simulink model "XFLUID04_reference"  (R2025a)
settings: Solver=ode23t  StartTime=0  StopTime=20  MaxStep=0.02  RelTol=1e-3  AbsTol=1e-4  EnableMultiTasking=on
PreLoadFcn:
  | warning('off','Simulink:Commands:LoadMdlParameterizedLink');
PostLoadFcn:
  | warning off sm:compiler:topologyAnalysis:DanglingBlock
  | warning off Simulink:SL_SolverMaskedZC;
  | warning off Simulink:SL_SolverIgnoredZCBracketing;
  | warning off Simulink:Engine:SolverMinStepNonlinearIterWarnForDAE;
  | warning off simscape:compiler:sli:init:SolverNotRecommended
  | warning off Simulink:Engine:UsingDiscreteSolver
  | warning('off','sm:sli:setup:compile:LocalSolverNotSupported')
  | warning off physmod:simscape:compiler:sli:init:SolverNotRecommended
  | warning off sm:sli:visualization:ModelRefNotSupported
  | warning off Simulink:modelReference:ProtectedModelCallbackLostWarning
StartFcn:
  | tic;
StopFcn:
  | Elapsed_Sim_Time = toc;
  | disp(['Elapsed Sim Time = ' num2str(Elapsed_Sim_Time)]);
undefined symbols (not defined in the file): actuator_hs_b, actuator_hs_k, lift_target_mm, Local, motion_start_s, motor_damping, pressure_step_offset_s, ramp_duration_s, Scissor_Lift_Param, supply_pressure_bar, supply_pressure_step_fraction, target_hold_s, X, Y, Z
libraries: fl_lib x108, sm_lib x41, Scissor_Parts_Lib x24, nesl_utility x9, SimscapeFluids_lib x2, Custom_lib x2, slpidlib x1, fl_ps_legacy_lib x1, simulink x1, ee_lib x1, Motor_Lib x1, sdl_lib x1
(part 3 of 3)

== system XFLUID04_reference/Load/Scissor/Base/Platform ==
  Block R : Scissor_Parts_Lib/Block  L=Scissor_Lift_Param.Upper_Platform.Length  W=Scissor_Lift_Param.Upper_Platform.Width  H=Scissor_Lift_Param.Upper_Platform.Height  z_ori=Local +Z  rho=Scissor_Lift_Param.Upper_Platform.Density  clr=Scissor_Lift_Param.Upper_Platform.Color  opc=Scissor_Lift_Param.Upper_Platform.Opacity
  Transform Orientation : sm_lib/Frames and Transforms/Rigid Transform  RotationMethod=StandardAxis  FollAlignAxisA=+X  BaseAlignAxisA=+Y  FollAlignAxisB=+Y  BaseAlignAxisB=+Z  RotationStandardAxis=+X  RotationAngle=90  RotationAngleUnits=deg  RotationArbitraryAxis=[0 0 1]  RotationSequenceAxes=FollowerAxes  RotationSequence=XYX  RotationSequenceAngles=[0 0 0]  RotationSequenceAnglesUnits=deg  RotationMatrix=[1 0 0; 0 1 0; 0 0 1]  Quaternion=[1 0 0 0]  TranslationMethod=None  TranslationCartesianOffset=[0 0 0]  TranslationCartesianOffsetUnits=m  TranslationStandardAxis=+X  TranslationStandardOffset=0  TranslationStandardOffsetUnits=m  TranslationROffset=0  TranslationROffsetUnits=m  TranslationThetaOffset=0  TranslationThetaOffsetUnits=deg  TranslationZOffset=0  TranslationZOffsetUnits=m
  Transform Platform CG : sm_lib/Frames and Transforms/Rigid Transform  RotationMethod=StandardAxis  FollAlignAxisA=+X  BaseAlignAxisA=+Y  FollAlignAxisB=+Y  BaseAlignAxisB=+Z  RotationStandardAxis=+Y  RotationAngle=90  RotationAngleUnits=deg  RotationArbitraryAxis=[0 0 1]  RotationSequenceAxes=FollowerAxes  RotationSequence=XYX  RotationSequenceAngles=[0 0 0]  RotationSequenceAnglesUnits=deg  RotationMatrix=[1 0 0; 0 1 0; 0 0 1]  Quaternion=[1 0 0 0]  TranslationMethod=StandardAxis  TranslationCartesianOffset=[0 0 0]  TranslationCartesianOffsetUnits=cm  TranslationStandardAxis=-X  TranslationStandardOffset=Scissor_Lift_Param.Link.Length  TranslationStandardOffsetUnits=cm  TranslationROffset=0  TranslationROffsetUnits=m  TranslationThetaOffset=0  TranslationThetaOffsetUnits=deg  TranslationZOffset=0  TranslationZOffsetUnits=m
  Transform Platform CP : sm_lib/Frames and Transforms/Rigid Transform  RotationMethod=None  FollAlignAxisA=+X  BaseAlignAxisA=+Y  FollAlignAxisB=+Y  BaseAlignAxisB=+Z  RotationStandardAxis=+Y  RotationAngle=0  RotationAngleUnits=deg  RotationArbitraryAxis=[0 0 1]  RotationSequenceAxes=FollowerAxes  RotationSequence=XYX  RotationSequenceAngles=[0 0 0]  RotationSequenceAnglesUnits=deg  RotationMatrix=[1 0 0; 0 1 0; 0 0 1]  Quaternion=[1 0 0 0]  TranslationMethod=Cartesian  TranslationCartesianOffset=[0 -Scissor_Lift_Param.Upper_Platform.Height/2 0]  TranslationCartesianOffsetUnits=cm  TranslationStandardAxis=-Y  TranslationStandardOffset=Scissor_Lift_Param.Roller.Roller_Radius  TranslationStandardOffsetUnits=cm  TranslationROffset=0  TranslationROffsetUnits=m  TranslationThetaOffset=0  TranslationThetaOffsetUnits=deg  TranslationZOffset=0  TranslationZOffsetUnits=m
  S : PMIOPort  Side=Right
  W : PMIOPort  Port=2  Side=Left
  connections:
  Block R/LConn1 -- Transform Platform CG/RConn1
  Transform Platform CP/RConn1 -- Transform Orientation/RConn1 -- Transform Platform CG/LConn1
  Transform Orientation/LConn1 -- W/RConn1
  Transform Platform CP/LConn1 -- S/RConn1

== system XFLUID04_reference/Load/Scissor/Base/Rear Shaft ==
  Blocks L : Scissor_Parts_Lib/Base Blocks  block_length=Scissor_Lift_Param.Base_Block.Length  block_width=Scissor_Lift_Param.Base_Block.Width  block_height=Scissor_Lift_Param.Base_Block.Height  shaft_radius=Scissor_Lift_Param.Roller.Shaft_Radius  shaft_length=Scissor_Lift_Param.Roller.Shaft_Length  material_density=Scissor_Lift_Param.Base_Block.Density  material_color=Scissor_Lift_Param.Base_Block.Color  material_opacity=Scissor_Lift_Param.Base_Block.Opacity
  Blocks R : Scissor_Parts_Lib/Base Blocks  block_length=Scissor_Lift_Param.Base_Block.Length  block_width=Scissor_Lift_Param.Base_Block.Width  block_height=Scissor_Lift_Param.Base_Block.Height  shaft_radius=Scissor_Lift_Param.Roller.Shaft_Radius  shaft_length=Scissor_Lift_Param.Roller.Shaft_Length  material_density=Scissor_Lift_Param.Base_Block.Density  material_color=Scissor_Lift_Param.Base_Block.Color  material_opacity=Scissor_Lift_Param.Base_Block.Opacity
  Shaft L : Scissor_Parts_Lib/Shaft  L=Scissor_Lift_Param.Base_Act_Shaft.Length/2  r=Scissor_Lift_Param.Base_Act_Shaft.Radius  theta=0  z_ori=Local +Z  Ro=Scissor_Lift_Param.Base_Act_Shaft.Density  clr=Scissor_Lift_Param.Base_Act_Shaft.Color  opc=Scissor_Lift_Param.Base_Act_Shaft.Opacity
  Shaft R : Scissor_Parts_Lib/Shaft  L=Scissor_Lift_Param.Base_Act_Shaft.Length/2  r=Scissor_Lift_Param.Base_Act_Shaft.Radius  theta=0  z_ori=Local +Z  Ro=Scissor_Lift_Param.Base_Act_Shaft.Density  clr=Scissor_Lift_Param.Base_Act_Shaft.Color  opc=Scissor_Lift_Param.Base_Act_Shaft.Opacity
  Transform Base Shaft : sm_lib/Frames and Transforms/Rigid Transform  RotationMethod=None  FollAlignAxisA=+X  BaseAlignAxisA=+Y  FollAlignAxisB=+Y  BaseAlignAxisB=+Z  RotationStandardAxis=+Y  RotationAngle=0  RotationAngleUnits=deg  RotationArbitraryAxis=[0 0 1]  RotationSequenceAxes=FollowerAxes  RotationSequence=XYX  RotationSequenceAngles=[0 0 0]  RotationSequenceAnglesUnits=deg  RotationMatrix=[1 0 0; 0 1 0; 0 0 1]  Quaternion=[1 0 0 0]  TranslationMethod=Cartesian  TranslationCartesianOffset=[0 -Scissor_Lift_Param.Base_Block.Height/2 0]  TranslationCartesianOffsetUnits=cm  TranslationStandardAxis=-Y  TranslationStandardOffset=Scissor_Lift_Param.Roller.Roller_Radius  TranslationStandardOffsetUnits=cm  TranslationROffset=0  TranslationROffsetUnits=m  TranslationThetaOffset=0  TranslationThetaOffsetUnits=deg  TranslationZOffset=0  TranslationZOffsetUnits=m
  Transform C to L : sm_lib/Frames and Transforms/Rigid Transform  RotationMethod=None  FollAlignAxisA=+X  BaseAlignAxisA=+Y  FollAlignAxisB=+Y  BaseAlignAxisB=+Z  RotationStandardAxis=+X  RotationAngle=90  RotationAngleUnits=deg  RotationArbitraryAxis=[0 0 1]  RotationSequenceAxes=FollowerAxes  RotationSequence=XYX  RotationSequenceAngles=[0 0 0]  RotationSequenceAnglesUnits=deg  RotationMatrix=[1 0 0; 0 1 0; 0 0 1]  Quaternion=[1 0 0 0]  TranslationMethod=StandardAxis  TranslationCartesianOffset=[0 0 0]  TranslationCartesianOffsetUnits=cm  TranslationStandardAxis=+Z  TranslationStandardOffset=Scissor_Lift_Param.Link_Separation.Outer_Outer/2  TranslationStandardOffsetUnits=cm  TranslationROffset=0  TranslationROffsetUnits=m  TranslationThetaOffset=0  TranslationThetaOffsetUnits=deg  TranslationZOffset=0  TranslationZOffsetUnits=m
  Transform C to R : sm_lib/Frames and Transforms/Rigid Transform  RotationMethod=None  FollAlignAxisA=+X  BaseAlignAxisA=+Y  FollAlignAxisB=+Y  BaseAlignAxisB=+Z  RotationStandardAxis=+X  RotationAngle=90  RotationAngleUnits=deg  RotationArbitraryAxis=[0 0 1]  RotationSequenceAxes=FollowerAxes  RotationSequence=XYX  RotationSequenceAngles=[0 0 0]  RotationSequenceAnglesUnits=deg  RotationMatrix=[1 0 0; 0 1 0; 0 0 1]  Quaternion=[1 0 0 0]  TranslationMethod=StandardAxis  TranslationCartesianOffset=[0 0 0]  TranslationCartesianOffsetUnits=cm  TranslationStandardAxis=-Z  TranslationStandardOffset=Scissor_Lift_Param.Link_Separation.Outer_Outer/2  TranslationStandardOffsetUnits=cm  TranslationROffset=0  TranslationROffsetUnits=m  TranslationThetaOffset=0  TranslationThetaOffsetUnits=deg  TranslationZOffset=0  TranslationZOffsetUnits=m
  R : PMIOPort  Side=Right
  P : PMIOPort  Port=2  Side=Left
  connections:
  Transform C to R/LConn1 -- Transform Base Shaft/RConn1 -- Transform C to L/LConn1 -- P/RConn1
  Blocks L/LConn1 -- Transform C to L/RConn1
  Shaft R/RConn1 -- Transform Base Shaft/LConn1 -- Shaft L/LConn1 -- R/RConn1
  Blocks R/LConn1 -- Transform C to R/RConn1

== system XFLUID04_reference/Load/Scissor/Inner Links/Link Connect ==
  Transform Outer FC : sm_lib/Frames and Transforms/Rigid Transform  RotationMethod=None  FollAlignAxisA=+X  BaseAlignAxisA=+Y  FollAlignAxisB=+Y  BaseAlignAxisB=+Z  RotationStandardAxis=+Z  RotationAngle=0  RotationAngleUnits=deg  RotationArbitraryAxis=[0 0 1]  RotationSequenceAxes=FollowerAxes  RotationSequence=XYX  RotationSequenceAngles=[0 0 0]  RotationSequenceAnglesUnits=deg  RotationMatrix=[1 0 0; 0 1 0; 0 0 1]  Quaternion=[1 0 0 0]  TranslationMethod=StandardAxis  TranslationCartesianOffset=[0 0 0]  TranslationCartesianOffsetUnits=cm  TranslationStandardAxis=+Z  TranslationStandardOffset=Scissor_Lift_Param.Link_Separation.Inner_Inner/2  TranslationStandardOffsetUnits=cm  TranslationROffset=0  TranslationROffsetUnits=m  TranslationThetaOffset=0  TranslationThetaOffsetUnits=deg  TranslationZOffset=0  TranslationZOffsetUnits=m
  Transform Outer FL : sm_lib/Frames and Transforms/Rigid Transform  RotationMethod=None  FollAlignAxisA=+X  BaseAlignAxisA=+Y  FollAlignAxisB=+Y  BaseAlignAxisB=+Z  RotationStandardAxis=+Z  RotationAngle=0  RotationAngleUnits=deg  RotationArbitraryAxis=[0 0 1]  RotationSequenceAxes=FollowerAxes  RotationSequence=XYX  RotationSequenceAngles=[0 0 0]  RotationSequenceAnglesUnits=deg  RotationMatrix=[1 0 0; 0 1 0; 0 0 1]  Quaternion=[1 0 0 0]  TranslationMethod=StandardAxis  TranslationCartesianOffset=[0 0 0]  TranslationCartesianOffsetUnits=cm  TranslationStandardAxis=+Z  TranslationStandardOffset=Scissor_Lift_Param.Link_Separation.Inner_Inner/2  TranslationStandardOffsetUnits=cm  TranslationROffset=0  TranslationROffsetUnits=m  TranslationThetaOffset=0  TranslationThetaOffsetUnits=deg  TranslationZOffset=0  TranslationZOffsetUnits=m
  L : PMIOPort  Side=Right
  C : PMIOPort  Port=2  Side=Left
  R : PMIOPort  Port=3  Side=Right
  connections:
  Transform Outer FL/LConn1 -- C/RConn1 -- Transform Outer FC/RConn1
  Transform Outer FC/LConn1 -- R/RConn1
  Transform Outer FL/RConn1 -- L/RConn1

== system XFLUID04_reference/Load/Scissor/Inner Links/Rollers ==
  Roller L : Scissor_Parts_Lib/Base Roller  roller_length=Scissor_Lift_Param.Roller.Roller_Length  roller_radius=Scissor_Lift_Param.Roller.Roller_Radius  shaft_length=Scissor_Lift_Param.Roller.Shaft_Length  shaft_radius=Scissor_Lift_Param.Roller.Shaft_Radius  material_density=Scissor_Lift_Param.Roller.Density  material_color=Scissor_Lift_Param.Roller.Color  material_opacity=Scissor_Lift_Param.Roller.Opacity
  Roller R : Scissor_Parts_Lib/Base Roller  roller_length=Scissor_Lift_Param.Roller.Roller_Length  roller_radius=Scissor_Lift_Param.Roller.Roller_Radius  shaft_length=Scissor_Lift_Param.Roller.Shaft_Length  shaft_radius=Scissor_Lift_Param.Roller.Shaft_Radius  material_density=Scissor_Lift_Param.Roller.Density  material_color=Scissor_Lift_Param.Roller.Color  material_opacity=Scissor_Lift_Param.Roller.Opacity
  Transform C to L : sm_lib/Frames and Transforms/Rigid Transform  RotationMethod=None  FollAlignAxisA=+X  BaseAlignAxisA=+Y  FollAlignAxisB=+Y  BaseAlignAxisB=+Z  RotationStandardAxis=+X  RotationAngle=90  RotationAngleUnits=deg  RotationArbitraryAxis=[0 0 1]  RotationSequenceAxes=FollowerAxes  RotationSequence=XYX  RotationSequenceAngles=[0 0 0]  RotationSequenceAnglesUnits=deg  RotationMatrix=[1 0 0; 0 1 0; 0 0 1]  Quaternion=[1 0 0 0]  TranslationMethod=StandardAxis  TranslationCartesianOffset=[0 0 0]  TranslationCartesianOffsetUnits=cm  TranslationStandardAxis=+Z  TranslationStandardOffset=Scissor_Lift_Param.Link_Separation.Inner_Inner/2  TranslationStandardOffsetUnits=cm  TranslationROffset=0  TranslationROffsetUnits=m  TranslationThetaOffset=0  TranslationThetaOffsetUnits=deg  TranslationZOffset=0  TranslationZOffsetUnits=m
  Transform C to R : sm_lib/Frames and Transforms/Rigid Transform  RotationMethod=None  FollAlignAxisA=+X  BaseAlignAxisA=+Y  FollAlignAxisB=+Y  BaseAlignAxisB=+Z  RotationStandardAxis=+X  RotationAngle=90  RotationAngleUnits=deg  RotationArbitraryAxis=[0 0 1]  RotationSequenceAxes=FollowerAxes  RotationSequence=XYX  RotationSequenceAngles=[0 0 0]  RotationSequenceAnglesUnits=deg  RotationMatrix=[1 0 0; 0 1 0; 0 0 1]  Quaternion=[1 0 0 0]  TranslationMethod=StandardAxis  TranslationCartesianOffset=[0 0 0]  TranslationCartesianOffsetUnits=cm  TranslationStandardAxis=-Z  TranslationStandardOffset=Scissor_Lift_Param.Link_Separation.Inner_Inner/2  TranslationStandardOffsetUnits=cm  TranslationROffset=0  TranslationROffsetUnits=m  TranslationThetaOffset=0  TranslationThetaOffsetUnits=deg  TranslationZOffset=0  TranslationZOffsetUnits=m
  Transform Lower P : sm_lib/Frames and Transforms/Rigid Transform  RotationMethod=StandardAxis  FollAlignAxisA=+X  BaseAlignAxisA=+Y  FollAlignAxisB=+Y  BaseAlignAxisB=+Z  RotationStandardAxis=+Y  RotationAngle=-90  RotationAngleUnits=deg  RotationArbitraryAxis=[0 0 1]  RotationSequenceAxes=FollowerAxes  RotationSequence=XYX  RotationSequenceAngles=[0 0 0]  RotationSequenceAnglesUnits=deg  RotationMatrix=[1 0 0; 0 1 0; 0 0 1]  Quaternion=[1 0 0 0]  TranslationMethod=Cartesian  TranslationCartesianOffset=[0 Scissor_Lift_Param.Base_Block.Height/2 0]  TranslationCartesianOffsetUnits=cm  TranslationStandardAxis=-Y  TranslationStandardOffset=Scissor_Lift_Param.Roller.Roller_Radius  TranslationStandardOffsetUnits=cm  TranslationROffset=0  TranslationROffsetUnits=m  TranslationThetaOffset=0  TranslationThetaOffsetUnits=deg  TranslationZOffset=0  TranslationZOffsetUnits=m
  S : PMIOPort  Side=Right
  LP : PMIOPort  Port=2  Side=Left
  connections:
  Roller L/RConn1 -- Transform C to L/RConn1
  Transform C to L/LConn1 -- Transform C to R/LConn1 -- Transform Lower P/RConn1 -- S/RConn1
  Roller R/RConn1 -- Transform C to R/RConn1
  Transform Lower P/LConn1 -- LP/RConn1

== system XFLUID04_reference/Load/Scissor/Inner Links/Shaft Actuator ==
  Shaft L : Scissor_Parts_Lib/Shaft  L=Scissor_Lift_Param.Link_Act_Shaft.Length/2  r=Scissor_Lift_Param.Link_Act_Shaft.Radius  theta=0  z_ori=Local +Z  Ro=Scissor_Lift_Param.Link_Act_Shaft.Density  clr=Scissor_Lift_Param.Colors.Yellow  opc=Scissor_Lift_Param.Link_Act_Shaft.Opacity
  Shaft R : Scissor_Parts_Lib/Shaft  L=Scissor_Lift_Param.Link_Act_Shaft.Length/2  r=Scissor_Lift_Param.Link_Act_Shaft.Radius  theta=0  z_ori=Local +Z  Ro=Scissor_Lift_Param.Link_Act_Shaft.Density  clr=Scissor_Lift_Param.Colors.Yellow  opc=Scissor_Lift_Param.Link_Act_Shaft.Opacity
  Transform Act Shaft : sm_lib/Frames and Transforms/Rigid Transform  RotationMethod=None  FollAlignAxisA=+X  BaseAlignAxisA=+Y  FollAlignAxisB=+Y  BaseAlignAxisB=+Z  RotationStandardAxis=+X  RotationAngle=90  RotationAngleUnits=deg  RotationArbitraryAxis=[0 0 1]  RotationSequenceAxes=FollowerAxes  RotationSequence=XYX  RotationSequenceAngles=[0 0 0]  RotationSequenceAnglesUnits=deg  RotationMatrix=[1 0 0; 0 1 0; 0 0 1]  Quaternion=[1 0 0 0]  TranslationMethod=StandardAxis  TranslationCartesianOffset=[0 0 0]  TranslationCartesianOffsetUnits=cm  TranslationStandardAxis=-X  TranslationStandardOffset=Scissor_Lift_Param.Link_Act_Shaft.Offset  TranslationStandardOffsetUnits=cm  TranslationROffset=0  TranslationROffsetUnits=m  TranslationThetaOffset=0  TranslationThetaOffsetUnits=deg  TranslationZOffset=0  TranslationZOffsetUnits=m
  Act : PMIOPort  Side=Right
  UP : PMIOPort  Port=2  Side=Left
  connections:
  Shaft R/RConn1 -- Shaft L/LConn1 -- Transform Act Shaft/RConn1 -- Act/RConn1
  Transform Act Shaft/LConn1 -- UP/RConn1

== system XFLUID04_reference/Load/Scissor/Outer Links/Rollers ==
  Roller L : Scissor_Parts_Lib/Base Roller  roller_length=Scissor_Lift_Param.Roller.Roller_Length  roller_radius=Scissor_Lift_Param.Roller.Roller_Radius  shaft_length=Scissor_Lift_Param.Roller.Shaft_Length  shaft_radius=Scissor_Lift_Param.Roller.Shaft_Radius  material_density=Scissor_Lift_Param.Roller.Density  material_color=Scissor_Lift_Param.Roller.Color  material_opacity=Scissor_Lift_Param.Roller.Opacity
  Roller R : Scissor_Parts_Lib/Base Roller  roller_length=Scissor_Lift_Param.Roller.Roller_Length  roller_radius=Scissor_Lift_Param.Roller.Roller_Radius  shaft_length=Scissor_Lift_Param.Roller.Shaft_Length  shaft_radius=Scissor_Lift_Param.Roller.Shaft_Radius  material_density=Scissor_Lift_Param.Roller.Density  material_color=Scissor_Lift_Param.Roller.Color  material_opacity=Scissor_Lift_Param.Roller.Opacity
  Transform C to L : sm_lib/Frames and Transforms/Rigid Transform  RotationMethod=None  FollAlignAxisA=+X  BaseAlignAxisA=+Y  FollAlignAxisB=+Y  BaseAlignAxisB=+Z  RotationStandardAxis=+X  RotationAngle=90  RotationAngleUnits=deg  RotationArbitraryAxis=[0 0 1]  RotationSequenceAxes=FollowerAxes  RotationSequence=XYX  RotationSequenceAngles=[0 0 0]  RotationSequenceAnglesUnits=deg  RotationMatrix=[1 0 0; 0 1 0; 0 0 1]  Quaternion=[1 0 0 0]  TranslationMethod=StandardAxis  TranslationCartesianOffset=[0 0 0]  TranslationCartesianOffsetUnits=cm  TranslationStandardAxis=+Z  TranslationStandardOffset=Scissor_Lift_Param.Link_Separation.Outer_Outer/2  TranslationStandardOffsetUnits=cm  TranslationROffset=0  TranslationROffsetUnits=m  TranslationThetaOffset=0  TranslationThetaOffsetUnits=deg  TranslationZOffset=0  TranslationZOffsetUnits=m
  Transform C to R : sm_lib/Frames and Transforms/Rigid Transform  RotationMethod=None  FollAlignAxisA=+X  BaseAlignAxisA=+Y  FollAlignAxisB=+Y  BaseAlignAxisB=+Z  RotationStandardAxis=+X  RotationAngle=90  RotationAngleUnits=deg  RotationArbitraryAxis=[0 0 1]  RotationSequenceAxes=FollowerAxes  RotationSequence=XYX  RotationSequenceAngles=[0 0 0]  RotationSequenceAnglesUnits=deg  RotationMatrix=[1 0 0; 0 1 0; 0 0 1]  Quaternion=[1 0 0 0]  TranslationMethod=StandardAxis  TranslationCartesianOffset=[0 0 0]  TranslationCartesianOffsetUnits=cm  TranslationStandardAxis=-Z  TranslationStandardOffset=Scissor_Lift_Param.Link_Separation.Outer_Outer/2  TranslationStandardOffsetUnits=cm  TranslationROffset=0  TranslationROffsetUnits=m  TranslationThetaOffset=0  TranslationThetaOffsetUnits=deg  TranslationZOffset=0  TranslationZOffsetUnits=m
  Transform Upper P : sm_lib/Frames and Transforms/Rigid Transform  RotationMethod=StandardAxis  FollAlignAxisA=+X  BaseAlignAxisA=+Y  FollAlignAxisB=+Y  BaseAlignAxisB=+Z  RotationStandardAxis=+Y  RotationAngle=-90  RotationAngleUnits=deg  RotationArbitraryAxis=[0 0 1]  RotationSequenceAxes=FollowerAxes  RotationSequence=XYX  RotationSequenceAngles=[0 0 0]  RotationSequenceAnglesUnits=deg  RotationMatrix=[1 0 0; 0 1 0; 0 0 1]  Quaternion=[1 0 0 0]  TranslationMethod=Cartesian  TranslationCartesianOffset=[0 -Scissor_Lift_Param.Base_Block.Height/2 0]  TranslationCartesianOffsetUnits=cm  TranslationStandardAxis=-Y  TranslationStandardOffset=Scissor_Lift_Param.Roller.Roller_Radius  TranslationStandardOffsetUnits=cm  TranslationROffset=0  TranslationROffsetUnits=m  TranslationThetaOffset=0  TranslationThetaOffsetUnits=deg  TranslationZOffset=0  TranslationZOffsetUnits=m
  UP : PMIOPort  Side=Right
  S : PMIOPort  Port=2  Side=Left
  connections:
  Transform C to R/LConn1 -- Transform Upper P/RConn1 -- Transform C to L/LConn1 -- S/RConn1
  Roller L/RConn1 -- Transform C to L/RConn1
  Transform Upper P/LConn1 -- UP/RConn1
  Roller R/RConn1 -- Transform C to R/RConn1

== system XFLUID04_reference/Load/Scissor/Outer Links/Shaft ==
  Transform Outer FC : sm_lib/Frames and Transforms/Rigid Transform  RotationMethod=None  FollAlignAxisA=+X  BaseAlignAxisA=+Y  FollAlignAxisB=+Y  BaseAlignAxisB=+Z  RotationStandardAxis=+Z  RotationAngle=0  RotationAngleUnits=deg  RotationArbitraryAxis=[0 0 1]  RotationSequenceAxes=FollowerAxes  RotationSequence=XYX  RotationSequenceAngles=[0 0 0]  RotationSequenceAnglesUnits=deg  RotationMatrix=[1 0 0; 0 1 0; 0 0 1]  Quaternion=[1 0 0 0]  TranslationMethod=StandardAxis  TranslationCartesianOffset=[0 0 0]  TranslationCartesianOffsetUnits=cm  TranslationStandardAxis=+Z  TranslationStandardOffset=Scissor_Lift_Param.Link_Separation.Outer_Outer/2  TranslationStandardOffsetUnits=cm  TranslationROffset=0  TranslationROffsetUnits=m  TranslationThetaOffset=0  TranslationThetaOffsetUnits=deg  TranslationZOffset=0  TranslationZOffsetUnits=m
  Transform Outer FL : sm_lib/Frames and Transforms/Rigid Transform  RotationMethod=None  FollAlignAxisA=+X  BaseAlignAxisA=+Y  FollAlignAxisB=+Y  BaseAlignAxisB=+Z  RotationStandardAxis=+Z  RotationAngle=0  RotationAngleUnits=deg  RotationArbitraryAxis=[0 0 1]  RotationSequenceAxes=FollowerAxes  RotationSequence=XYX  RotationSequenceAngles=[0 0 0]  RotationSequenceAnglesUnits=deg  RotationMatrix=[1 0 0; 0 1 0; 0 0 1]  Quaternion=[1 0 0 0]  TranslationMethod=StandardAxis  TranslationCartesianOffset=[0 0 0]  TranslationCartesianOffsetUnits=cm  TranslationStandardAxis=+Z  TranslationStandardOffset=Scissor_Lift_Param.Link_Separation.Outer_Outer/2  TranslationStandardOffsetUnits=cm  TranslationROffset=0  TranslationROffsetUnits=m  TranslationThetaOffset=0  TranslationThetaOffsetUnits=deg  TranslationZOffset=0  TranslationZOffsetUnits=m
  L : PMIOPort  Side=Right
  C : PMIOPort  Port=2  Side=Left
  R : PMIOPort  Port=3  Side=Right
  connections:
  Transform Outer FL/RConn1 -- L/RConn1
  Transform Outer FC/LConn1 -- R/RConn1
  Transform Outer FC/RConn1 -- C/RConn1 -- Transform Outer FL/LConn1

== system XFLUID04_reference/Load/Scissor/Upper Platform/Blocks ==
  Blocks L : Scissor_Parts_Lib/Base Blocks  block_length=Scissor_Lift_Param.Base_Block.Length  block_width=Scissor_Lift_Param.Base_Block.Width  block_height=Scissor_Lift_Param.Base_Block.Height  shaft_radius=Scissor_Lift_Param.Roller.Shaft_Radius  shaft_length=Scissor_Lift_Param.Roller.Shaft_Length  material_density=Scissor_Lift_Param.Base_Block.Density  material_color=Scissor_Lift_Param.Base_Block.Color  material_opacity=Scissor_Lift_Param.Base_Block.Opacity
  Blocks R : Scissor_Parts_Lib/Base Blocks  block_length=Scissor_Lift_Param.Base_Block.Length  block_width=Scissor_Lift_Param.Base_Block.Width  block_height=Scissor_Lift_Param.Base_Block.Height  shaft_radius=Scissor_Lift_Param.Roller.Shaft_Radius  shaft_length=Scissor_Lift_Param.Roller.Shaft_Length  material_density=Scissor_Lift_Param.Base_Block.Density  material_color=Scissor_Lift_Param.Base_Block.Color  material_opacity=Scissor_Lift_Param.Base_Block.Opacity
  Transform C to L : sm_lib/Frames and Transforms/Rigid Transform  RotationMethod=None  FollAlignAxisA=+X  BaseAlignAxisA=+Y  FollAlignAxisB=+Y  BaseAlignAxisB=+Z  RotationStandardAxis=+X  RotationAngle=90  RotationAngleUnits=deg  RotationArbitraryAxis=[0 0 1]  RotationSequenceAxes=FollowerAxes  RotationSequence=XYX  RotationSequenceAngles=[0 0 0]  RotationSequenceAnglesUnits=deg  RotationMatrix=[1 0 0; 0 1 0; 0 0 1]  Quaternion=[1 0 0 0]  TranslationMethod=StandardAxis  TranslationCartesianOffset=[0 0 0]  TranslationCartesianOffsetUnits=cm  TranslationStandardAxis=+Z  TranslationStandardOffset=Scissor_Lift_Param.Link_Separation.Inner_Inner/2  TranslationStandardOffsetUnits=cm  TranslationROffset=0  TranslationROffsetUnits=m  TranslationThetaOffset=0  TranslationThetaOffsetUnits=deg  TranslationZOffset=0  TranslationZOffsetUnits=m
  Transform C to R : sm_lib/Frames and Transforms/Rigid Transform  RotationMethod=None  FollAlignAxisA=+X  BaseAlignAxisA=+Y  FollAlignAxisB=+Y  BaseAlignAxisB=+Z  RotationStandardAxis=+X  RotationAngle=90  RotationAngleUnits=deg  RotationArbitraryAxis=[0 0 1]  RotationSequenceAxes=FollowerAxes  RotationSequence=XYX  RotationSequenceAngles=[0 0 0]  RotationSequenceAnglesUnits=deg  RotationMatrix=[1 0 0; 0 1 0; 0 0 1]  Quaternion=[1 0 0 0]  TranslationMethod=StandardAxis  TranslationCartesianOffset=[0 0 0]  TranslationCartesianOffsetUnits=cm  TranslationStandardAxis=-Z  TranslationStandardOffset=Scissor_Lift_Param.Link_Separation.Inner_Inner/2  TranslationStandardOffsetUnits=cm  TranslationROffset=0  TranslationROffsetUnits=m  TranslationThetaOffset=0  TranslationThetaOffsetUnits=deg  TranslationZOffset=0  TranslationZOffsetUnits=m
  Transform Platform : sm_lib/Frames and Transforms/Rigid Transform  RotationMethod=None  FollAlignAxisA=+X  BaseAlignAxisA=+Y  FollAlignAxisB=+Y  BaseAlignAxisB=+Z  RotationStandardAxis=+Y  RotationAngle=0  RotationAngleUnits=deg  RotationArbitraryAxis=[0 0 1]  RotationSequenceAxes=FollowerAxes  RotationSequence=XYX  RotationSequenceAngles=[0 0 0]  RotationSequenceAnglesUnits=deg  RotationMatrix=[1 0 0; 0 1 0; 0 0 1]  Quaternion=[1 0 0 0]  TranslationMethod=Cartesian  TranslationCartesianOffset=[0 Scissor_Lift_Param.Base_Block.Height/2 0]  TranslationCartesianOffsetUnits=cm  TranslationStandardAxis=-Y  TranslationStandardOffset=Scissor_Lift_Param.Roller.Roller_Radius  TranslationStandardOffsetUnits=cm  TranslationROffset=0  TranslationROffsetUnits=m  TranslationThetaOffset=0  TranslationThetaOffsetUnits=deg  TranslationZOffset=0  TranslationZOffsetUnits=m
  UP : PMIOPort  Side=Right
  S : PMIOPort  Port=2  Side=Left
  connections:
  Transform Platform/LConn1 -- S/RConn1 -- Transform C to R/LConn1 -- Transform C to L/LConn1
  Transform Platform/RConn1 -- UP/RConn1
  Transform C to L/RConn1 -- Blocks L/RConn1
  Transform C to R/RConn1 -- Blocks R/RConn1
